simulink model "timespdr"  (R2018a)
settings: Solver=ode23  StartTime=0.0  StopTime=0.3  RelTol=1e-3
libraries: powerlib x11
settings Model: Creator=simlab2025  LastModifiedBy=simlab2025

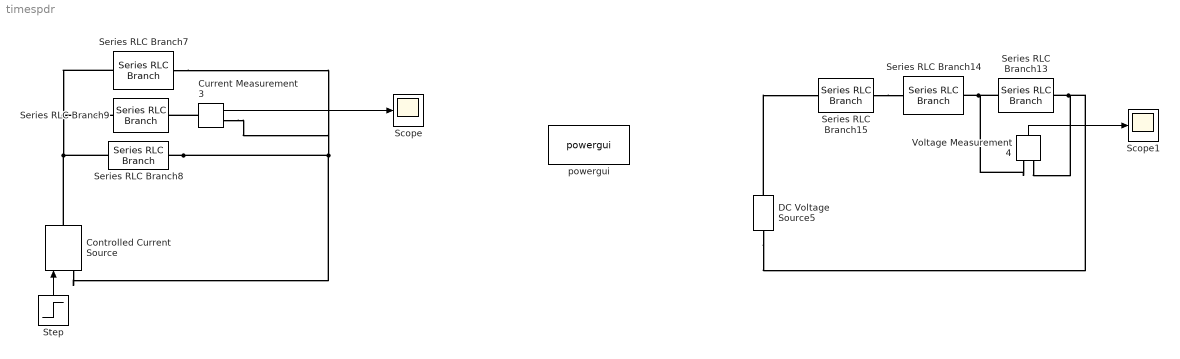
== system timespdr ==
  Controlled Current Source : powerlib/Electrical Sources/Controlled Current Source  Initialize=on  Source_Type=AC  Amplitude=0  Phase=0  Frequency=0  Measurements=None
  Current Measurement3 : powerlib/Measurements/Current Measurement  PhasorSimulation=off  OutputType=Complex  PSBequivalent=0
  DC Voltage Source5 : powerlib/Electrical Sources/DC Voltage Source  Amplitude=10  Measurements=None
  Scope : Scope
  Scope1 : Scope
  Series RLC Branch13 : powerlib/Elements/Series RLC Branch  LConnTagsString=__new0  RConnTagsString=__new0  BranchType=C  Resistance=20  Inductance=1  SetiL0=on  InitialCurrent=0  Capacitance=1e-4  Setx0=on  InitialVoltage=0  Measurements=None
  Series RLC Branch14 : powerlib/Elements/Series RLC Branch  LConnTagsString=__new0  RConnTagsString=__new0  BranchType=R  Resistance=20  Inductance=1  SetiL0=on  InitialCurrent=0  Capacitance=1e-6  Setx0=on  InitialVoltage=0  Measurements=None
  Series RLC Branch15 : powerlib/Elements/Series RLC Branch  LConnTagsString=__new0  RConnTagsString=__new0  BranchType=L  Resistance=200  Inductance=0.5  SetiL0=on  InitialCurrent=0  Capacitance=0  Setx0=off  InitialVoltage=0  Measurements=None
  Series RLC Branch7 : powerlib/Elements/Series RLC Branch  LConnTagsString=__new0  RConnTagsString=__new0  BranchType=C  Resistance=5  Inductance=1  SetiL0=on  InitialCurrent=0  Capacitance=1e-6  Setx0=on  InitialVoltage=0  Measurements=None
  Series RLC Branch8 : powerlib/Elements/Series RLC Branch  LConnTagsString=__new0  RConnTagsString=__new0  BranchType=R  Resistance=20000  Inductance=1  SetiL0=on  InitialCurrent=0  Capacitance=0  Setx0=off  InitialVoltage=0  Measurements=None
  Series RLC Branch9 : powerlib/Elements/Series RLC Branch  LConnTagsString=__new0  RConnTagsString=__new0  BranchType=L  Resistance=200  Inductance=75  SetiL0=on  InitialCurrent=0  Capacitance=0  Setx0=off  InitialVoltage=0  Measurements=None
  Step : Step  Time=0.01  After=10  SampleTime=0
  Voltage Measurement4 : powerlib/Measurements/Voltage Measurement  PhasorSimulation=off  OutputType=Complex  PSBequivalent=0
  powergui : powerlib/powergui  Priority=1  SimulationMode=Discrete  SampleTime=50e-6  frequency=60  Iterations=50  frequencyindice=0  Pbase=100e6  ErrMax=1e-4  UnitsV=kV  UnitsW=MW  buscounter=0  FunctionMessages=off  echomessages=off  EnableUseOfTLC=off  CurrentSourceSwitches=off  DisableSnubberDevices=off  DisableRonSwitches=off  DisableVfSwitches=off  DisplayEquations=off  SolverType=Tustin/Backward Euler (TBE)  Interpol=off  ExternalGateDelay=off  methode=off  Ts=100  x0status=blocks  SPID=on  SwTol=0  HookPort=off  RestoreLinks=warning  ResistiveCurrentMeasurement=off  Frange=[0:2:500]  Ylog=off  Xlog=on  ShowGrid=off  save=off  variable=ZData  structure=0  ZoomFFT=off  StartTime=0.0  cycles=1  DisplayStyle=1  fundamental=60  FreqAxis=off  MaxFrequency=1000  frequencyindicesteady=1  RmsSteady=1  display=off
  wires:
  Current Measurement3/1 -> Scope/1
  Step/1 -> Controlled Current Source/1
  Voltage Measurement4/1 -> Scope1/1
  connections:
  Series RLC Branch8/RConn1 -- Series RLC Branch7/LConn1 -- Current Measurement3/RConn1 -- Controlled Current Source/LConn1
  Series RLC Branch9/LConn1 -- Series RLC Branch7/RConn1 -- Series RLC Branch8/LConn1 -- Controlled Current Source/RConn1
  Current Measurement3/LConn1 -- Series RLC Branch9/RConn1
  Series RLC Branch14/LConn1 -- Series RLC Branch13/LConn1 -- Voltage Measurement4/LConn1
  Series RLC Branch13/RConn1 -- DC Voltage Source5/LConn1 -- Voltage Measurement4/LConn2
  Series RLC Branch15/RConn1 -- Series RLC Branch14/RConn1
  DC Voltage Source5/RConn1 -- Series RLC Branch15/LConn1
